simulink library "Motor_Lib"  (R2024a)
settings: Solver=VariableStepAuto  StartTime=0.0  StopTime=10.0  RelTol=1e-3
undefined symbols (not defined in the file): YBT_Par
libraries: fl_lib x13, nesl_utility x5, ee_lib x3, sdl_lib x1
Description:
  | Copyright 2017-2024 The MathWorks, Inc.
settings Model: Creator=smiller  LastModifiedBy=smiller
settings SolverCC: AlgebraicLoopSolver=TrustRegion
settings DataIOCC: ReturnWorkspaceOutputs=off
settings OptimizationCC: ReuseModelBlockBuffer=off
settings DebuggingCC: UnconnectedInputMsg=warning  UnconnectedOutputMsg=warning  UnconnectedLineMsg=warning  PregeneratedLibrarySubsystemCodeDiagnostic=none  ArithmeticOperatorsInVariantConditions=warning
settings ModelReferenceCC: EnableRefExpFcnMdlSchedulingChecks=on
settings SFSimCC: SimUseLocalCustomCode=off  CustomCodeUndefinedFunction=UseInterfaceOnly
settings RTWCC: RTWUseLocalCustomCode=off  GPUComputeCapability=3.5  DLArmComputeVersion=19.05
settings CodeAppCC: StateflowObjectComments=on

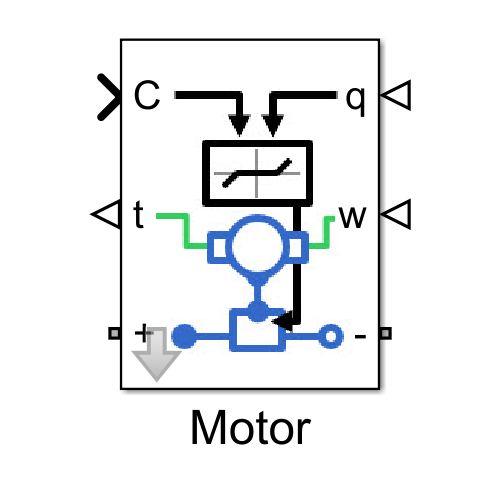
[thumbnail: Simulink's stored preview of the top-level diagram]
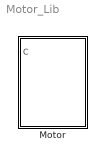
== system Motor_Lib ==
  Motor : Subsystem  RequirementInfo={} %GIDa_59e01a2d_ff26_4594_a2c7_77f0f29cc504  VariantControl=Motor  mask{r_motor=YBT_Par.Bicep.Motor.R, l_motor=YBT_Par.Bicep.Motor.L, k_motor=1/YBT_Par.Bicep.Motor.K, i_motor_noLoad=YBT_Par.Bicep.Motor.no_load_i, v_supply=YBT_Par.Battery.v, gear_ratio=YBT_Par.Bicep.Motor.gr, friction_visc=YBT_Par.Bicep.Motor.friction, ctrl_deadZone=YBT_Par.Control.Dead_Band}
      mask prompts: r_motor "Armature Resistance (Ohm)"; l_motor "Armature Inductance (H)"; k_motor "Torque Constant (N*(m/A))"; i_motor_noLoad "No-Load Current (A)"; v_supply "Supply Voltage (V)"; gear_ratio "Gear Ratio"; friction_visc "Viscous Friction (N*m/(rad/s))"; ctrl_deadZone "Dead Zone (deg)"
      mask DialogControl Container4 Prompt: Electrical
      mask DialogControl Container5 Prompt: Mechanical
      mask DialogControl Container6 Prompt: Control
      mask Display: image('youBot_Arm_Motor_JointIntf_IMAGE.jpg');

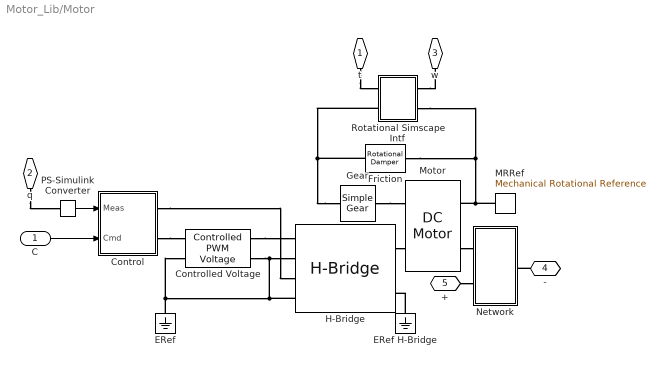
== system Motor_Lib/Motor ==
  C : Inport  RequirementInfo={} %GIDa_368bb575_4ebf_43b9_b4ea_49c24a069202
  Control : Subsystem  RequirementInfo={} %GIDa_1ec0417b_7c76_4050_9d46_00f29d0701f9
  Controlled Voltage : ee_lib/Integrated Circuits/Controlled PWM Voltage  RequirementInfo={} %GIDa_73809545_7df6_434d_99db_e1e4c007496a  F=1000 Hz  TD=0 s  pulse_width_offset=0 s  pulse_min=0 s  pwm_or_av=2  event_type=1  sample_time=1e-6 s  Vmin=0 V  Vmax=5 V  Vm=5 V  u_min=0  u_max=1
  ERef : fl_lib/Electrical/Electrical Elements/Electrical Reference  RequirementInfo={} %GIDa_13c4472f_b89b_482f_9ffb_b40e92d1d3b6
  ERef H-Bridge : fl_lib/Electrical/Electrical Elements/Electrical Reference  RequirementInfo={} %GIDa_45275578_1c20_43d7_90b2_7bfacb70d4e2
  Friction : fl_lib/Mechanical/Rotational Elements/Rotational Damper  RequirementInfo={} %GIDa_95420ff3_9dcf_4e97_b73e_38948f5541ef  D=friction_visc N*m/(rad/s)  w_specify=off  w_priority=None  w=0 rad/s  w_nominal_specify=off  w_nominal_value=1  w_nominal_unit=rad/s  t_specify=off  t_priority=None  t=0 N*m  t_nominal_specify=off  t_nominal_value=1  t_nominal_unit=N*m
  Gear : sdl_lib/Gears/Simple Gear  RequirementInfo={} %GIDa_08249044_1c97_412f_9f83_d43ac5b48ee2  ratio=gear_ratio  rotation_direction=3-2*(1)  enable_faults=simscape.enum.onoff.off  efficiency_fault=0.05  fault_angles=pi / 12 rad  friction_model=1  T_noload=0.1 N*m  T_nom=5 N*m  efficiency_nom=0.8  efficiency=0.8  temperature_TLU=[ 280 300 320 ] K  load_TLU=[ 1 5 10 ] N*m  efficiency_TLU=[ 0.95 0.9 0.85 ]  efficiency_TLU2=[ 0.85 0.8 0.75; 0.95 0.9 0.85; 0.85 0.8 0.7 ]  w_thr=0.01 rad/s  pwr_thr=0.001 W  enable_backlash=false  hardstop_model=simscape.enum.hardstop.smooth  backlash_distance=1e-3 mm  r_base=0.1 m  transition=1e-4 mm  backlash_stiffness=1e7 N/m  backlash_damping=1e6 N*s/m  coeff_rest=0  v_tol=0.001 m/s  f_tol=0 N  mu_visc=[ 0 0 ] N*m/(rad/s)  thermal_mass=50 J/K  temperature_specify=off  temperature_priority=High  temperature=300 K  temperature_nominal_specify=off  temperature_nominal_value=1  temperature_nominal_unit=K  x_backlash_specify=off  x_backlash_priority=None  x_backlash=0 mm  x_backlash_nominal_specify=off  x_backlash_nominal_value=1  x_backlash_nominal_unit=mm  f_hardstop_specify=off  f_hardstop_priority=None  f_hardstop=0 N  f_hardstop_nominal_specify=off  f_hardstop_nominal_value=1  f_hardstop_nominal_unit=N  v_backlash_specify=off  v_backlash_priority=None  v_backlash=0 m/s  v_backlash_nominal_specify=off  v_backlash_nominal_value=1  v_backlash_nominal_unit=m/s
  H-Bridge : ee_lib/Semiconductors & Converters/Converters/H-Bridge  RequirementInfo={} %GIDa_2d920dd3_d64f_4e64_9840_7eeb6e433ba1  supply_ports=ee.enum.supply_ports.hidesupply  pwm_or_av=2  regenerative_braking_mode=2  discontinuous=0  freewheeling_mode=1  Rload=10 Ohm  Lload=1e-5 H  F=10 kHz  Venable=2.5 V  Vmax=5.0 V  Vreverse=2.5 V  Vbrake=2.5 V  Vm=24 V  Ron=0.1 Ohm  Don=0.05 Ohm  Goff=1e-6 S  Tmeas=298.15 K  Ron2=0.1 Ohm  Don2=0.05 Ohm  Tmeas2=398.15 K  thermal_mass=100 J/K  initial_temperature=298.15 K
  MRRef : fl_lib/Mechanical/Rotational Elements/Mechanical Rotational Reference  RequirementInfo={} %GIDa_f2f8a82a_ccb9_438c_b8d8_d7fb0f28210b
  Motor : ee_lib/Electromechanical/Brushed Motors/DC Motor  RequirementInfo={} %GIDa_e8fd8f66_930b_46bd_9aeb_7cabcba805e7  field_option=ee.enum.field_option.pm  Rf=100 Ohm  Lf=1 H  Laf=0.15 H  If0=0 A  parameterization=1  Ra=r_motor Ohm  La=l_motor H  emf_or_torque=2  Kv=YBT_Par.Pivot.Motor.K V/rpm  Ki=k_motor N*m/A  T_stall=2.4e-4 N*m  w_max=1.91e+4 rpm  w_rated=1.5e+4 rpm  P_rated=0.08 W  V_rated=1.5 V  lam_param=2  i_noload=i_motor_noLoad A  V_i_noload=v_supply V  J=0 g*cm^2  lam=0 N*m/(rad/s)  speed0=0 rpm  enable_fault_armature=simscape.enum.onoff.off  rev_faulted=1 / 3  G_faulted_armature=1e-5 S  fault_trigger_armature=ee.enum.faults.faultTrigger.temporal  t_fault_armature=1 s  max_permissible_current_armature=inf A  t_fail_on_current_armature=1 s  enable_fault_field=simscape.enum.onoff.off  G_faulted_field=1e-5 S  fault_trigger_field=ee.enum.faults.faultTrigger.temporal  t_fault_field=1 s  max_permissible_current_field=inf A  t_fail_on_current_field=1 s  fault_action=simscape.enum.assert.action.none  alpha=3.93e-3 1/K  Tmeas=25 degC  thermal_mass=100 J/K  initial_temperature=25 degC
  Network : Subsystem  RequirementInfo={} %GIDa_9fee18e3_a948_413b_b883_e16fb674c0c0
  PS-Simulink Converter : nesl_utility/PS-Simulink Converter  RequirementInfo={} %GIDa_097674be_c2d9_46a2_88c8_91219fb03945  PhysicalDomain=network_engine_domain  SubClassName=ps_output  LeftPortType=input  RightPortType=output  PseudoPeriodic=off  Frequencies=[]  VectorFormat=1-D array  Unit=deg  AffineConversion=off
  Rotational Simscape Intf : Subsystem  RequirementInfo={} %GIDa_20a566a3_cdb1_4068_bc1b_4a204c2bcbb6
  t : PMIOPort  RequirementInfo={} %GIDa_a4b14222_3c31_477c_b014_3f812253a7d1  Side=Left
  q : PMIOPort  RequirementInfo={} %GIDa_573a934d_9532_4ee2_a8de_871da8711231  Port=2  Side=Right
  w : PMIOPort  RequirementInfo={} %GIDa_6a3eaa94_65d6_407b_b016_769070f6a746  Port=3  Side=Right
  - : PMIOPort  RequirementInfo={} %GIDa_ba051fe7_3f5b_4fff_b5df_531125b4f6cf  Port=4  Side=Right
  + : PMIOPort  RequirementInfo={} %GIDa_03fc6ed1_1d24_43d2_9ab2_d0402432e792  Port=5  Side=Left
  wires:
  PS-Simulink Converter/1 -> Control/1(Meas)
  C/1 -> Control/2(Cmd)
  connections:
  Rotational Simscape Intf/RConn1 -- w/RConn1
  q/RConn1 -- PS-Simulink Converter/LConn1
  +/RConn1 -- Network/LConn2
  -/RConn1 -- Network/RConn1
  Motor/RConn1 -- Network/LConn1
  ERef H-Bridge/LConn1 -- H-Bridge/RConn2
  Control/RConn1 -- H-Bridge/LConn3
  Control/RConn2 -- Controlled Voltage/LConn1
  H-Bridge/RConn1 -- Motor/LConn1
  H-Bridge/LConn4 -- Controlled Voltage/LConn2 -- ERef/LConn1 -- H-Bridge/LConn2 -- Controlled Voltage/RConn2
  Controlled Voltage/RConn1 -- H-Bridge/LConn1
  t/RConn1 -- Rotational Simscape Intf/LConn1
  Rotational Simscape Intf/RConn2 -- Friction/RConn1 -- Motor/RConn2 -- MRRef/LConn1
  Gear/LConn1 -- Motor/LConn2
  Gear/RConn1 -- Rotational Simscape Intf/LConn2 -- Friction/LConn1

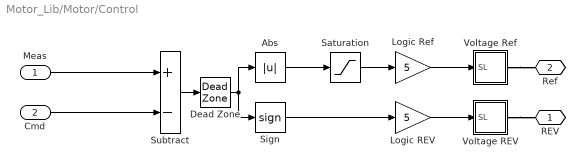
== system Motor_Lib/Motor/Control ==
  Meas : Inport  RequirementInfo={} %GIDa_619c2803_28d3_4ef7_ba70_833e220e126d
  Cmd : Inport  RequirementInfo={} %GIDa_cedc12fc_cc18_42d0_9a71_21d4f8b9a5ca  Port=2
  Abs : Abs  RequirementInfo={} %GIDa_d0313f18_77fc_4469_88ee_421a3cb03dd3  ZeroCross=off  SaturateOnIntegerOverflow=off
  Dead Zone : DeadZone  RequirementInfo={} %GIDa_8c142244_20db_463a_b94f_674c218bd698  LowerValue=-ctrl_deadZone  UpperValue=ctrl_deadZone  ZeroCross=off
  Logic REV : Gain  RequirementInfo={} %GIDa_b932483c_9411_4fcb_821f_6d68825134f0  Gain=5
  Logic Ref : Gain  RequirementInfo={} %GIDa_11f4073f_f2f5_4fa6_a867_14315e93e3df  Gain=5
  Saturation : Saturate  UpperLimit=1  LowerLimit=0  ZeroCross=off
  Sign : Signum  RequirementInfo={} %GIDa_d20f7fe8_60b8_4a21_b668_3ad824d4ede9  ZeroCross=off
  Subtract : Sum  RequirementInfo={} %GIDa_19bf5a43_019a_4db9_b97f_957f1fcc13e1  Inputs=+-
  Voltage REV : Subsystem  RequirementInfo={} %GIDa_c0e87e75_602b_4cdc_bd7f_8168c58f4b38
  Voltage Ref : Subsystem  RequirementInfo={} %GIDa_8f8c4948_8993_460a_8a8e_45d690a1b1f5
  REV : PMIOPort  RequirementInfo={} %GIDa_bf5c9ce0_d82a_4963_bef4_f9b0d83d66de  Side=Right
  Ref : PMIOPort  RequirementInfo={} %GIDa_1cf45b29_5f52_4f47_a585_a1bd10a239a7  Port=2  Side=Right
  wires:
  Dead Zone/1 -> Sign/1, Abs/1
  Subtract/1 -> Dead Zone/1
  Logic Ref/1 -> Voltage Ref/1(SL)
  Cmd/1 -> Subtract/2
  Logic REV/1 -> Voltage REV/1(SL)
  Sign/1 -> Logic REV/1
  Abs/1 -> Saturation/1
  Meas/1 -> Subtract/1
  Saturation/1 -> Logic Ref/1
  connections:
  Voltage REV/RConn1 -- REV/RConn1
  Voltage Ref/RConn1 -- Ref/RConn1

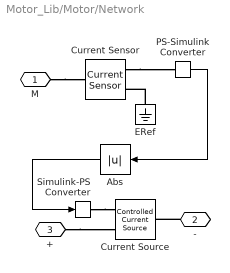
== system Motor_Lib/Motor/Network ==
  Abs : Abs  ZeroCross=off  SaturateOnIntegerOverflow=off
  Current Sensor : fl_lib/Electrical/Electrical Sensors/Current Sensor  RequirementInfo={} %GIDa_513c3105_2bac_45e4_b484_9e853d23afd7
  Current Source : fl_lib/Electrical/Electrical Sources/Controlled Current Source  RequirementInfo={} %GIDa_94a24adf_c038_4ce1_83ad_37f20f638e14
  ERef : fl_lib/Electrical/Electrical Elements/Electrical Reference
  PS-Simulink Converter : nesl_utility/PS-Simulink Converter  PhysicalDomain=network_engine_domain  SubClassName=ps_output  LeftPortType=input  RightPortType=output  PseudoPeriodic=off  Frequencies=[]  VectorFormat=1-D array  Unit=1  AffineConversion=off
  Simulink-PS Converter : nesl_utility/Simulink-PS Converter  PhysicalDomain=network_engine_domain  SubClassName=ps_input  LeftPortType=input  RightPortType=output  PseudoPeriodic=off  Frequencies=[]  NoiseDistribution=none  NoiseParameters=[]  Unit=1  AffineConversion=off  FilteringAndDerivatives=zero  SimscapeFilterOrder=1  InputFilterTimeConstant=0.005  UdotUserProvided=1
  " M" : PMIOPort  RequirementInfo={} %GIDa_84871c60_653c_4020_b9b8_d9b6ede8c9f6  Side=Left
  - : PMIOPort  RequirementInfo={} %GIDa_c912cfdd_b223_4c72_a577_976fa4621da7  Port=2  Side=Right
  + : PMIOPort  RequirementInfo={} %GIDa_bf626ff5_1ed8_4472_be8d_8f3179a83c03  Port=3  Side=Left
  wires:
  PS-Simulink Converter/1 -> Abs/1
  Abs/1 -> Simulink-PS Converter/1
  connections:
  -/RConn1 -- Current Source/LConn1
  +/RConn1 -- Current Source/RConn2
  Current Sensor/RConn1 -- PS-Simulink Converter/LConn1
  " M"/RConn1 -- Current Sensor/LConn1
  ERef/LConn1 -- Current Sensor/RConn2
  Simulink-PS Converter/RConn1 -- Current Source/RConn1

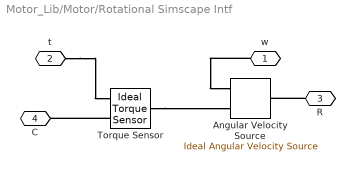
== system Motor_Lib/Motor/Rotational Simscape Intf ==
  Angular Velocity Source : fl_lib/Mechanical/Mechanical Sources/Ideal Angular Velocity Source  RequirementInfo={} %GIDa_9c63d25c_cbc1_48c9_8ca4_1c1f53bf651e
  Torque Sensor : fl_lib/Mechanical/Mechanical Sensors/Ideal Torque Sensor  RequirementInfo={} %GIDa_cf1090dc_72bf_4751_af0a_ba0ab775e595
  w : PMIOPort  RequirementInfo={} %GIDa_f25d5e0a_0e94_4d54_ac21_7ad0e7ab5701  Side=Right
  t : PMIOPort  RequirementInfo={} %GIDa_028763a7_4726_4672_beaf_1abf56a90cfd  Port=2  Side=Left
  R : PMIOPort  RequirementInfo={} %GIDa_22d96cb3_e01c_43f5_a1b0_795c055d4914  Port=3  Side=Left
  C : PMIOPort  RequirementInfo={} %GIDa_120a4565_964d_4dd8_b46f_0df667ed0ae0  Port=4  Side=Right
  connections:
  w/RConn1 -- Angular Velocity Source/RConn1
  t/RConn1 -- Torque Sensor/RConn2
  Torque Sensor/LConn1 -- Angular Velocity Source/RConn2
  R/RConn1 -- Angular Velocity Source/LConn1
  Torque Sensor/RConn1 -- C/RConn1

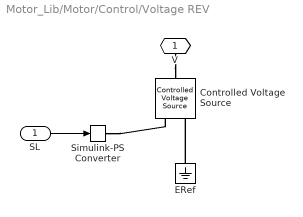
== system Motor_Lib/Motor/Control/Voltage REV ==
  SL : Inport  RequirementInfo={} %GIDa_dea8ea81_1710_4fb8_ba02_6f2c02265479
  Controlled Voltage Source : fl_lib/Electrical/Electrical Sources/Controlled Voltage Source  RequirementInfo={} %GIDa_18b8d214_2427_4381_a540_d572da4e9001
  ERef : fl_lib/Electrical/Electrical Elements/Electrical Reference  RequirementInfo={} %GIDa_462338b2_4d7f_47c7_89f7_87b59660760b
  Simulink-PS Converter : nesl_utility/Simulink-PS Converter  RequirementInfo={} %GIDa_0fb8daf5_cf0e_41aa_bdfd_c463d772de6d  PhysicalDomain=network_engine_domain  SubClassName=ps_input  LeftPortType=input  RightPortType=output  PseudoPeriodic=off  Frequencies=[]  NoiseDistribution=none  NoiseParameters=[]  Unit=V  AffineConversion=off  FilteringAndDerivatives=zero  SimscapeFilterOrder=1  InputFilterTimeConstant=0.005  UdotUserProvided=0
  V : PMIOPort  RequirementInfo={} %GIDa_c42b8280_047e_43ce_ada1_0ab47814a1ff  Side=Right
  wires:
  SL/1 -> Simulink-PS Converter/1
  connections:
  ERef/LConn1 -- Controlled Voltage Source/RConn2
  V/RConn1 -- Controlled Voltage Source/LConn1
  Simulink-PS Converter/RConn1 -- Controlled Voltage Source/RConn1

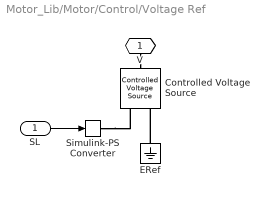
== system Motor_Lib/Motor/Control/Voltage Ref ==
  SL : Inport  RequirementInfo={} %GIDa_419a7471_849d_441c_84b1_4e25bcdc027c
  Controlled Voltage Source : fl_lib/Electrical/Electrical Sources/Controlled Voltage Source  RequirementInfo={} %GIDa_6e64d9cc_3e6c_4d3a_a6fc_3228a91425c7
  ERef : fl_lib/Electrical/Electrical Elements/Electrical Reference  RequirementInfo={} %GIDa_884cea57_6d0e_4e6b_b934_7eb0c59af366
  Simulink-PS Converter : nesl_utility/Simulink-PS Converter  RequirementInfo={} %GIDa_7c09949d_fb09_4c67_b267_9eeb2ab661fd  PhysicalDomain=network_engine_domain  SubClassName=ps_input  LeftPortType=input  RightPortType=output  PseudoPeriodic=off  Frequencies=[]  NoiseDistribution=none  NoiseParameters=[]  Unit=V  AffineConversion=off  FilteringAndDerivatives=zero  SimscapeFilterOrder=1  InputFilterTimeConstant=0.005  UdotUserProvided=0
  V : PMIOPort  RequirementInfo={} %GIDa_06de9ff4_dfb2_4b63_b424_d78d422e5b2d  Side=Right
  wires:
  SL/1 -> Simulink-PS Converter/1
  connections:
  Simulink-PS Converter/RConn1 -- Controlled Voltage Source/RConn1
  V/RConn1 -- Controlled Voltage Source/LConn1
  ERef/LConn1 -- Controlled Voltage Source/RConn2
